simulink model "aircraft_6dof_gp"  (R2025b)
settings: Solver=VariableStepAuto  StartTime=0.0  StopTime=10.0  RelTol=1e-3
settings Model: Creator=HP  LastModifiedBy=HP

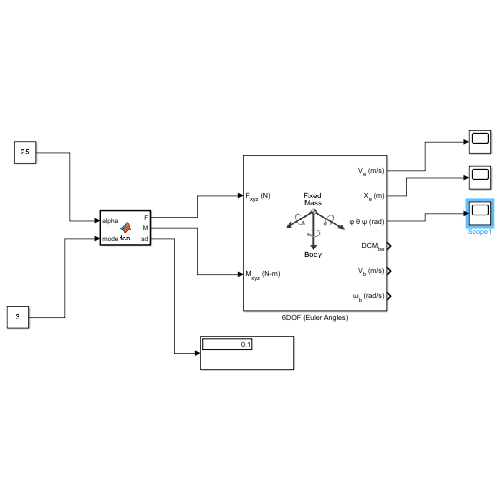
[thumbnail: Simulink's stored preview of the top-level diagram]
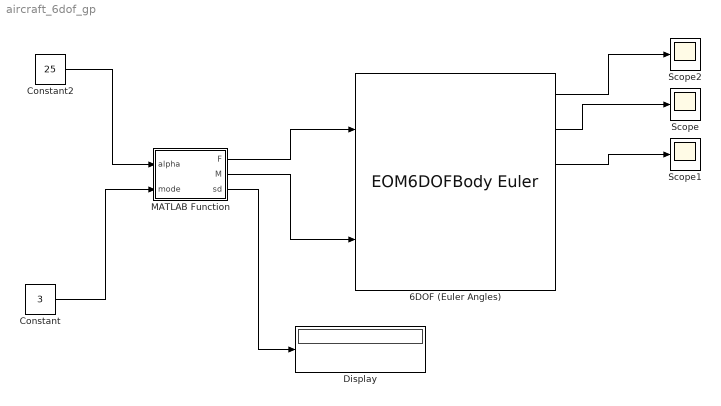
== system aircraft_6dof_gp ==
  6DOF (Euler Angles) : EOM6DOFBodyEuler  Vm_0=[30 0 0]  mass_0=5
  Constant : Constant  Value=3
  Constant2 : Constant  Value=25
  Display : Display
  MATLAB Function : MATLAB Function  TreatAsAtomicUnit=on
  Scope : Scope
      settings: ActiveDisplayYMinimum=-754.24501640625067  ActiveDisplayYMaximum=385.68952265625018
  Scope1 : Scope
      settings: ActiveDisplayYMinimum=-1  ActiveDisplayYMaximum=1
  Scope2 : Scope
      settings: ActiveDisplayYMinimum=-147.80660156250013  ActiveDisplayYMaximum=49.756289062500016  DataLoggingVariableName=ScopeData2
  wires:
  6DOF (Euler Angles)/2 -> Scope/1
  6DOF (Euler Angles)/1 -> Scope2/1
  6DOF (Euler Angles)/3 -> Scope1/1
  Constant2/1 -> MATLAB Function/1(alpha)
  MATLAB Function/1(F) -> 6DOF (Euler Angles)/1
  MATLAB Function/2(M) -> 6DOF (Euler Angles)/2
  MATLAB Function/3(sd) -> Display/1
  Constant/1 -> MATLAB Function/2(mode)

== matlab function aircraft_6dof_gp/MATLAB Function ==
  data: alpha input; F output; M output; sd output; mode input
function [F, M, sd] = fcn(alpha, mode)
coder.extrinsic('gp_predict');
coder.extrinsic('lookup_predict');

% Aircraft numbers (docs/aircraft_assumptions.md)
rho  = 1.225;   % air density, kg/m3
V    = 30;      % airspeed, m/s
S    = 0.15;    % wing area, m2
mass = 5;       % kg
g    = 9.81;    % m/s2
mach = 0.1;     % Mach passed to the models
thr  = 0.00879; % locked uncertainty threshold

yg = zeros(1,3);
yl = zeros(1,3);
sd = 0;
[yg, sd] = gp_predict(alpha, mach);
yl = lookup_predict(alpha, mach);

% Choose the source of CL and CD
if mode == 1
    y = yl;                 % lookup only
elseif mode == 2
    y = yg;                 % GP only
else
    if sd > thr
        y = yl;             % GP unsure, use lookup
    else
        y = yg;             % GP sure, use GP
    end
end

q = 0.5 * rho * V^2 * S;

Lift   = q * y(1);
Drag   = q * y(2);
Weight = mass * g;

% NED axes: down is +z, so lift is -z and weight is +z
F = [-Drag; 0; -Lift + Weight];
M = [0; 0; 0];   % pitching moment off (no tail in this model)   
end
